simulink model "PID_Controller"  (R2026b)
settings: Solver=VariableStepAuto  StopTime=20.0
values from neighbouring files (symbols this model uses):
  g = 9.81    [init_dron.m]
  kd = m * 2 * zeta * wn    (= 14.4)    [init_dron.m]
  ki = 2    [init_dron.m]
  kp = m * wn^2    (= 24)    [init_dron.m]
  m = 1.5    [init_dron.m]
  u_max = 35    [init_dron.m]
  u_min = 0    [init_dron.m]
settings Model: Creator=Rodrigo  LastModifiedBy=Rodrigo

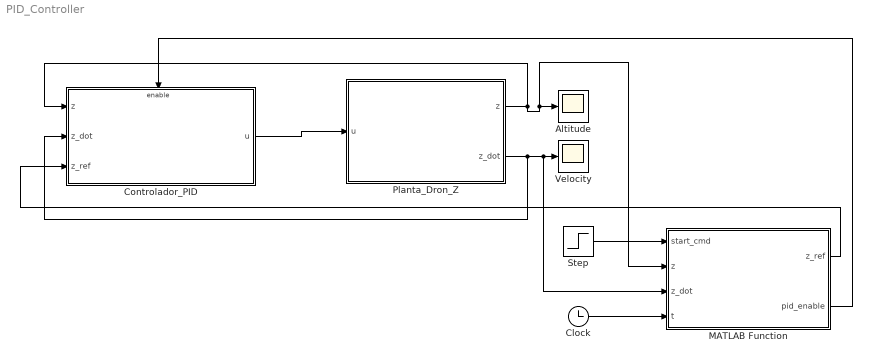
== system PID_Controller ==
  Altitude : Scope
      settings: ActiveDisplayYMinimum=-1.7591453694881327  ActiveDisplayYMaximum=11.40071394742589
  Clock : Clock
  Controlador_PID : Subsystem
  MATLAB Function : MATLAB Function  TreatAsAtomicUnit=on
  Planta_Dron_Z : Subsystem
  Step : Step  SampleTime=0
  Velocity : Scope
      settings: ActiveDisplayYMinimum=-13.392777675046576  ActiveDisplayYMaximum=12.624999075419179
  wires:
  Step/1 -> MATLAB Function/1(start_cmd)
  Controlador_PID/1(u) -> Planta_Dron_Z/1(u)
  Planta_Dron_Z/1(z) -> MATLAB Function/2(z), Altitude/1, Controlador_PID/1(z)
  Planta_Dron_Z/2(z_dot) -> MATLAB Function/3(z_dot), Velocity/1, Controlador_PID/2(z_dot)
  Clock/1 -> MATLAB Function/4(t)
  MATLAB Function/2(pid_enable) -> Controlador_PID/Enable
  MATLAB Function/1(z_ref) -> Controlador_PID/3(z_ref)

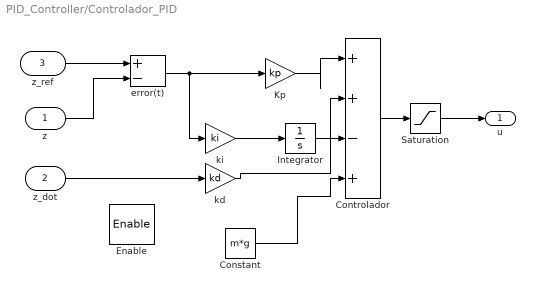
== system PID_Controller/Controlador_PID ==
  z : Inport
  z_dot : Inport  Port=2
  z_ref : Inport  Port=3
  Enable : EnablePort  StatesWhenEnabling=reset
  Constant : Constant  Value=m*g
  Controlador : Sum  Inputs=|++-+
  Integrator : Integrator  LimitOutput=on  UpperSaturationLimit=3  LowerSaturationLimit=-3
  Kp : Gain  Gain=kp
  Saturation : Saturate  UpperLimit=u_max  LowerLimit=u_min
  error(t) : Sum  Inputs=+-
  kd : Gain  Gain=kd
  ki : Gain  Gain=ki
  u : Outport  OutputWhenDisabled=reset  InitialOutput=0
  wires:
  z/1 -> error(t)/2
  z_ref/1 -> error(t)/1
  Kp/1 -> Controlador/1
  error(t)/1 -> ki/1, Kp/1
  Integrator/1 -> Controlador/2
  z_dot/1 -> kd/1
  kd/1 -> Controlador/3
  Controlador/1 -> Saturation/1
  Saturation/1 -> u/1
  ki/1 -> Integrator/1
  Constant/1 -> Controlador/4

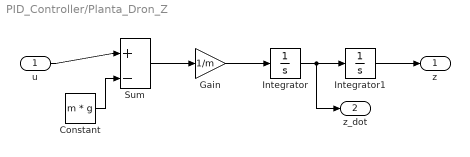
== system PID_Controller/Planta_Dron_Z ==
  u : Inport
  Constant : Constant  Value=m * g
  Gain : Gain  Gain=1/m
  Integrator : Integrator
  Integrator1 : Integrator  LimitOutput=on  LowerSaturationLimit=0
  Sum : Sum  Inputs=|+-
  z : Outport
  z_dot : Outport  Port=2
  wires:
  u/1 -> Sum/1
  Constant/1 -> Sum/2
  Sum/1 -> Gain/1
  Gain/1 -> Integrator/1
  Integrator/1 -> z_dot/1, Integrator1/1
  Integrator1/1 -> z/1

== matlab function PID_Controller/MATLAB Function ==
  settings: updateMethod=DISCRETE  sampleTime=0.1
  data: start_cmd input; z_ref output; z input; z_dot input; pid_enable output; t input
function [z_ref, pid_enable] = Supervisor_Mission(start_cmd, z, z_dot, t)

% parametros
Z_TAKEOFF = 10;
POS_TOL_HOVER = 0.15;
VEL_TOL_HOVER = 0.20;
HOVER_TIME = 5.0;

POS_TOL_LAND = 0.05;
VEL_TOL_LAND = 0.10;

% variables persistent
persistent estado
persistent t_inicio_hover

if isempty(estado)
    estado = 0;
    t_inicio_hover = 0;
end

% maquina de estados
switch estado
    case 0 % IDLE
        pid_enable = 0;
        z_ref = 0;

        if start_cmd == 1
            estado = 1;
        end
        
    case 1  % TAKEOFF
        pid_enable = 1;
        z_ref = Z_TAKEOFF;

        if abs(z-Z_TAKEOFF) < POS_TOL_HOVER && abs(z_dot) < VEL_TOL_HOVER
            estado = 2;
            t_inicio_hover = t;
        end
    
    case 2 % HOVER
        pid_enable = 1;
        z_ref = Z_TAKEOFF;

        if t >= t_inicio_hover + HOVER_TIME
            estado = 3;
        end

    case 3
        pid_enable = 1;
        z_ref = 0;

        if abs(z) < POS_TOL_LAND && abs(z_dot) < VEL_TOL_LAND
            pid_enable = 0;
            estado = 4;
        end

    case 4 % MISSION COMPLETE
        pid_enable = 0;
        z_ref = 0;

    otherwise
        pid_enable = 0;
        z_ref = 0;

end
end
